simulink model "SINGLE_STAR_TEN_LEG_AMB"  (R2025b)
settings: Solver=VariableStepAuto  StartTime=0.0  StopTime=0.008  MaxStep=1e-6  RelTol=1e-4
model workspace (MAT data in the model file):
  Ki = 47.1238898038
  Kp = 0.0235619449019
  L_w = 0.0005
  M = [0 0 0 0 0 0 1 0 0 0 0 0 ... (100 elements, 10x10)]
  R_w = 1
  T_stop = 0.008
  T_sw = 5e-05
  Ts_ctrl = 2.5e-05
  U_dc = 200
  duty = [0.51375 0.46375 0.49125 0.45875 0.53625 0.48625 0.54125 0.46875 0.46375 0.51875]
  f_c = 1500
  f_sw = 20000
  i_bias = 5
  i_ctrl = 1
  i_ctrl_by_dof = [1 1 1 1 1]
  i_ref = [5.5 4.5 5.5 4.5 5.5 4.5 5.5 4.5 5.5 4.5]
  phi = [0 4.5 -5.5 0 -6.5 9 -1 10 -4.5 -5.5 5.5]
  u = [5.5 4.5 5.5 4.5 5.5 4.5 5.5 4.5 5.5 4.5]
  wn_fb = 37699.1118431
  zeta_fb = 0.707
libraries: fl_lib x51, simulink x31, nesl_utility x31, ee_lib x21
(part 4 of 4)

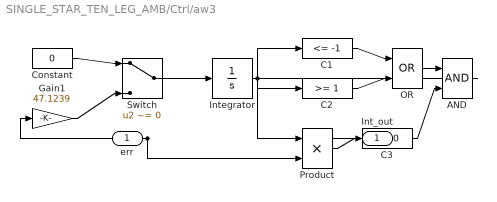
== system SINGLE_STAR_TEN_LEG_AMB/Ctrl/aw3 ==
  err : Inport
  AND : Logic  AllPortsSameDT=off  OutDataTypeStr=boolean
  C1 : simulink/Logic and Bit Operations/Compare To Constant  relop=<=  const=-1  OutDataTypeStr=boolean
  C2 : simulink/Logic and Bit Operations/Compare To Constant  relop=>=  const=1  OutDataTypeStr=boolean
  C3 : simulink/Logic and Bit Operations/Compare To Constant  relop=>=  const=0  OutDataTypeStr=boolean
  Constant : Constant  Value=0
  Gain1 : Gain  Gain=47.1239
  Integrator : Integrator  LimitOutput=on  UpperSaturationLimit=1  LowerSaturationLimit=-1
  OR : Logic  Operator=OR  AllPortsSameDT=off  OutDataTypeStr=boolean
  Product : Product
  Switch : Switch  Criteria=u2 ~= 0  SaturateOnIntegerOverflow=off  InputSameDT=off
  Int_out : Outport
  wires:
  err/1 -> Gain1/1, Product/2
  Constant/1 -> Switch/1
  Gain1/1 -> Switch/3
  Switch/1 -> Integrator/1
  Integrator/1 -> C1/1, C2/1, Product/1, Int_out/1
  C1/1 -> OR/1
  C2/1 -> OR/2
  Product/1 -> C3/1
  OR/1 -> AND/1
  C3/1 -> AND/2
  AND/1 -> Switch/2

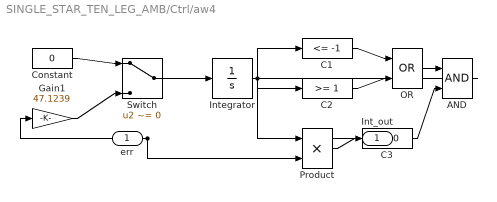
== system SINGLE_STAR_TEN_LEG_AMB/Ctrl/aw4 ==
  err : Inport
  AND : Logic  AllPortsSameDT=off  OutDataTypeStr=boolean
  C1 : simulink/Logic and Bit Operations/Compare To Constant  relop=<=  const=-1  OutDataTypeStr=boolean
  C2 : simulink/Logic and Bit Operations/Compare To Constant  relop=>=  const=1  OutDataTypeStr=boolean
  C3 : simulink/Logic and Bit Operations/Compare To Constant  relop=>=  const=0  OutDataTypeStr=boolean
  Constant : Constant  Value=0
  Gain1 : Gain  Gain=47.1239
  Integrator : Integrator  LimitOutput=on  UpperSaturationLimit=1  LowerSaturationLimit=-1
  OR : Logic  Operator=OR  AllPortsSameDT=off  OutDataTypeStr=boolean
  Product : Product
  Switch : Switch  Criteria=u2 ~= 0  SaturateOnIntegerOverflow=off  InputSameDT=off
  Int_out : Outport
  wires:
  err/1 -> Gain1/1, Product/2
  Constant/1 -> Switch/1
  Gain1/1 -> Switch/3
  Switch/1 -> Integrator/1
  Integrator/1 -> C1/1, C2/1, Product/1, Int_out/1
  C1/1 -> OR/1
  C2/1 -> OR/2
  Product/1 -> C3/1
  OR/1 -> AND/1
  C3/1 -> AND/2
  AND/1 -> Switch/2

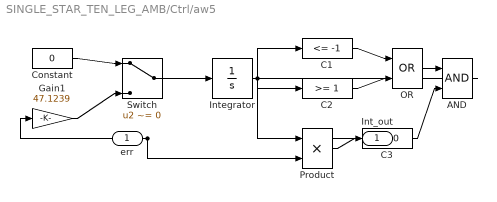
== system SINGLE_STAR_TEN_LEG_AMB/Ctrl/aw5 ==
  err : Inport
  AND : Logic  AllPortsSameDT=off  OutDataTypeStr=boolean
  C1 : simulink/Logic and Bit Operations/Compare To Constant  relop=<=  const=-1  OutDataTypeStr=boolean
  C2 : simulink/Logic and Bit Operations/Compare To Constant  relop=>=  const=1  OutDataTypeStr=boolean
  C3 : simulink/Logic and Bit Operations/Compare To Constant  relop=>=  const=0  OutDataTypeStr=boolean
  Constant : Constant  Value=0
  Gain1 : Gain  Gain=47.1239
  Integrator : Integrator  LimitOutput=on  UpperSaturationLimit=1  LowerSaturationLimit=-1
  OR : Logic  Operator=OR  AllPortsSameDT=off  OutDataTypeStr=boolean
  Product : Product
  Switch : Switch  Criteria=u2 ~= 0  SaturateOnIntegerOverflow=off  InputSameDT=off
  Int_out : Outport
  wires:
  err/1 -> Gain1/1, Product/2
  Constant/1 -> Switch/1
  Gain1/1 -> Switch/3
  Switch/1 -> Integrator/1
  Integrator/1 -> C1/1, C2/1, Product/1, Int_out/1
  C1/1 -> OR/1
  C2/1 -> OR/2
  Product/1 -> C3/1
  OR/1 -> AND/1
  C3/1 -> AND/2
  AND/1 -> Switch/2

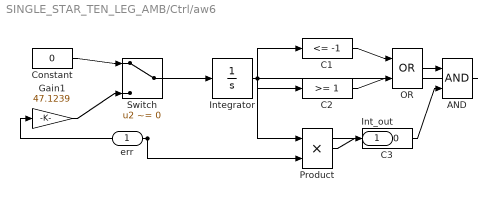
== system SINGLE_STAR_TEN_LEG_AMB/Ctrl/aw6 ==
  err : Inport
  AND : Logic  AllPortsSameDT=off  OutDataTypeStr=boolean
  C1 : simulink/Logic and Bit Operations/Compare To Constant  relop=<=  const=-1  OutDataTypeStr=boolean
  C2 : simulink/Logic and Bit Operations/Compare To Constant  relop=>=  const=1  OutDataTypeStr=boolean
  C3 : simulink/Logic and Bit Operations/Compare To Constant  relop=>=  const=0  OutDataTypeStr=boolean
  Constant : Constant  Value=0
  Gain1 : Gain  Gain=47.1239
  Integrator : Integrator  LimitOutput=on  UpperSaturationLimit=1  LowerSaturationLimit=-1
  OR : Logic  Operator=OR  AllPortsSameDT=off  OutDataTypeStr=boolean
  Product : Product
  Switch : Switch  Criteria=u2 ~= 0  SaturateOnIntegerOverflow=off  InputSameDT=off
  Int_out : Outport
  wires:
  err/1 -> Gain1/1, Product/2
  Constant/1 -> Switch/1
  Gain1/1 -> Switch/3
  Switch/1 -> Integrator/1
  Integrator/1 -> C1/1, C2/1, Product/1, Int_out/1
  C1/1 -> OR/1
  C2/1 -> OR/2
  Product/1 -> C3/1
  OR/1 -> AND/1
  C3/1 -> AND/2
  AND/1 -> Switch/2

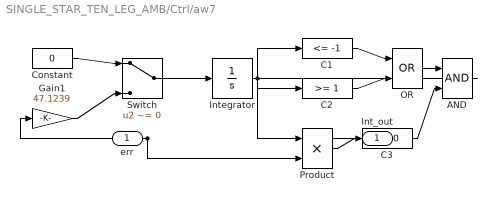
== system SINGLE_STAR_TEN_LEG_AMB/Ctrl/aw7 ==
  err : Inport
  AND : Logic  AllPortsSameDT=off  OutDataTypeStr=boolean
  C1 : simulink/Logic and Bit Operations/Compare To Constant  relop=<=  const=-1  OutDataTypeStr=boolean
  C2 : simulink/Logic and Bit Operations/Compare To Constant  relop=>=  const=1  OutDataTypeStr=boolean
  C3 : simulink/Logic and Bit Operations/Compare To Constant  relop=>=  const=0  OutDataTypeStr=boolean
  Constant : Constant  Value=0
  Gain1 : Gain  Gain=47.1239
  Integrator : Integrator  LimitOutput=on  UpperSaturationLimit=1  LowerSaturationLimit=-1
  OR : Logic  Operator=OR  AllPortsSameDT=off  OutDataTypeStr=boolean
  Product : Product
  Switch : Switch  Criteria=u2 ~= 0  SaturateOnIntegerOverflow=off  InputSameDT=off
  Int_out : Outport
  wires:
  err/1 -> Gain1/1, Product/2
  Constant/1 -> Switch/1
  Gain1/1 -> Switch/3
  Switch/1 -> Integrator/1
  Integrator/1 -> C1/1, C2/1, Product/1, Int_out/1
  C1/1 -> OR/1
  C2/1 -> OR/2
  Product/1 -> C3/1
  OR/1 -> AND/1
  C3/1 -> AND/2
  AND/1 -> Switch/2

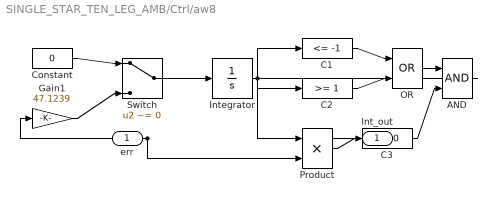
== system SINGLE_STAR_TEN_LEG_AMB/Ctrl/aw8 ==
  err : Inport
  AND : Logic  AllPortsSameDT=off  OutDataTypeStr=boolean
  C1 : simulink/Logic and Bit Operations/Compare To Constant  relop=<=  const=-1  OutDataTypeStr=boolean
  C2 : simulink/Logic and Bit Operations/Compare To Constant  relop=>=  const=1  OutDataTypeStr=boolean
  C3 : simulink/Logic and Bit Operations/Compare To Constant  relop=>=  const=0  OutDataTypeStr=boolean
  Constant : Constant  Value=0
  Gain1 : Gain  Gain=47.1239
  Integrator : Integrator  LimitOutput=on  UpperSaturationLimit=1  LowerSaturationLimit=-1
  OR : Logic  Operator=OR  AllPortsSameDT=off  OutDataTypeStr=boolean
  Product : Product
  Switch : Switch  Criteria=u2 ~= 0  SaturateOnIntegerOverflow=off  InputSameDT=off
  Int_out : Outport
  wires:
  err/1 -> Gain1/1, Product/2
  Constant/1 -> Switch/1
  Gain1/1 -> Switch/3
  Switch/1 -> Integrator/1
  Integrator/1 -> C1/1, C2/1, Product/1, Int_out/1
  C1/1 -> OR/1
  C2/1 -> OR/2
  Product/1 -> C3/1
  OR/1 -> AND/1
  C3/1 -> AND/2
  AND/1 -> Switch/2

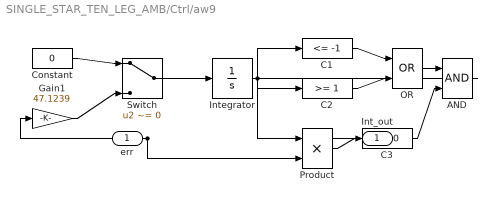
== system SINGLE_STAR_TEN_LEG_AMB/Ctrl/aw9 ==
  err : Inport
  AND : Logic  AllPortsSameDT=off  OutDataTypeStr=boolean
  C1 : simulink/Logic and Bit Operations/Compare To Constant  relop=<=  const=-1  OutDataTypeStr=boolean
  C2 : simulink/Logic and Bit Operations/Compare To Constant  relop=>=  const=1  OutDataTypeStr=boolean
  C3 : simulink/Logic and Bit Operations/Compare To Constant  relop=>=  const=0  OutDataTypeStr=boolean
  Constant : Constant  Value=0
  Gain1 : Gain  Gain=47.1239
  Integrator : Integrator  LimitOutput=on  UpperSaturationLimit=1  LowerSaturationLimit=-1
  OR : Logic  Operator=OR  AllPortsSameDT=off  OutDataTypeStr=boolean
  Product : Product
  Switch : Switch  Criteria=u2 ~= 0  SaturateOnIntegerOverflow=off  InputSameDT=off
  Int_out : Outport
  wires:
  err/1 -> Gain1/1, Product/2
  Constant/1 -> Switch/1
  Gain1/1 -> Switch/3
  Switch/1 -> Integrator/1
  Integrator/1 -> C1/1, C2/1, Product/1, Int_out/1
  C1/1 -> OR/1
  C2/1 -> OR/2
  Product/1 -> C3/1
  OR/1 -> AND/1
  C3/1 -> AND/2
  AND/1 -> Switch/2
